simulink model "acoustic_pursuit_loop"  (R2026b)
settings: Solver=ode4  StopTime=30  FixedStep=0.01
model workspace (MAT data in the model file):
  Pc = [-0.955361961697; -8.18538892611e-15; -1.20667677978e-16; -0.534217529105; -8.61310855498e-16; -1.23431548867; -0.21823206593; -8.91503756517e-15; 0.05; 0; 0; -0.00125; 0; 0.25; 0.5; 0.523598775598; 0.145; 1; 1.3962634016; 0.1; 1; 0.05; 2.4; 0.03; 0.1]
  Po = [1; 0; 0; 0; 0; 0; 1; 0; 0; 0; 0; 0.125; 1; 0; 0; 0.05; 0; 0; 1; 0; 0; 0.003125; 0.05; 0; 1; -0.05; 0; 0; 0; 0; 0; -0.053125; -0.05; 0; 0; 1; 0; 0; 1; 0; 0; 0; 0; 0; 0; 0.878680113902; -3.59557130076e-18; 3.54139223511e-16; 0.51922603514; 7.21443661026e-16; -2.65527818364e-18; 0.970658487238; 1.08350382663; -8.10062906002e-17; 1.38781881493; 1; 0; 0; 0; 0; 0; 1; 0; 0; 0; 0; 0.75; 1; 0; 0; 0.3; 0; 0; 1; 0; 0; 0.1125; 0.3; 0; 1; 0.00370925831023; -5.96618963202e-20; -5.96618963197e-20; 0.0207679892018; 9.21; 0.15; 0.261799387799]
  Ps = [1; 1; 0.436332312999; 0.436332312999; 0.01; 0.05; 0.1; 0; 0.5; 0; 0; 5.6; 0.5]
  Td = 0.3
  Td_obs = 0.25
  Tdw = 0.1
  Tm = 0.4
  Ts = 0.05
  tau_v = 0.2
  tau_w = 0.15
  v0 = 0.25
  wt = [0.3; 0]
  x0 = [1.1; 0; 0]
settings Model: Creator=Admin  LastModifiedBy=Admin

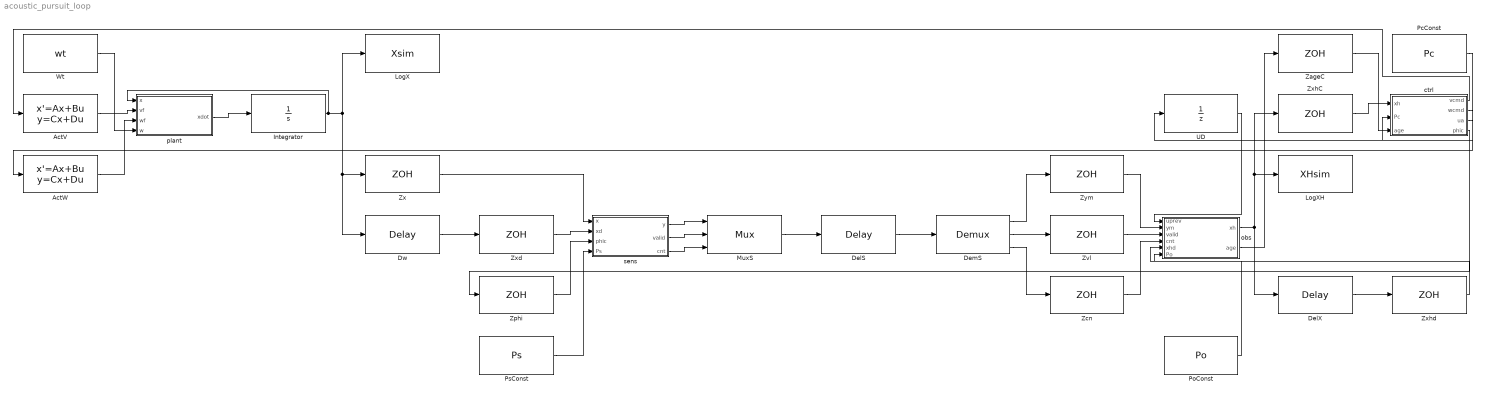
== system acoustic_pursuit_loop ==
  ActV : StateSpace  A=-1/tau_v  B=1/tau_v  D=0  InitialCondition=v0
  ActW : StateSpace  A=-1/tau_w  B=1/tau_w  D=0  InitialCondition=0
  DelS : TransportDelay  DelayTime=Td  InitialOutput=zeros(4,1)
  DelX : TransportDelay  DelayTime=Td_obs  InitialOutput=zeros(5,1)
  DemS : Demux  Outputs=[2 1 1]
  Dw : TransportDelay  DelayTime=Tdw  InitialOutput=x0
  Integrator : Integrator  InitialCondition=x0
  LogX : ToWorkspace  VariableName=Xsim  SampleTime=-1
  LogXH : ToWorkspace  VariableName=XHsim  SampleTime=-1
  MuxS : Mux  Inputs=3
  PcConst : Constant  Value=Pc
  PoConst : Constant  Value=Po
  PsConst : Constant  Value=Ps
  UD : UnitDelay  InitialCondition=[0;0]  SampleTime=Ts
  Wt : Constant  Value=wt
  ZageC : ZeroOrderHold  SampleTime=Ts
  Zcn : ZeroOrderHold  SampleTime=Ts
  Zphi : ZeroOrderHold  SampleTime=Tm
  Zvl : ZeroOrderHold  SampleTime=Ts
  Zx : ZeroOrderHold  SampleTime=Tm
  Zxd : ZeroOrderHold  SampleTime=Tm
  ZxhC : ZeroOrderHold  SampleTime=Ts
  Zxhd : ZeroOrderHold  SampleTime=Ts
  Zym : ZeroOrderHold  SampleTime=Ts
  ctrl : MATLAB Function  TreatAsAtomicUnit=on
  obs : MATLAB Function  TreatAsAtomicUnit=on
  plant : MATLAB Function  TreatAsAtomicUnit=on
  sens : MATLAB Function  TreatAsAtomicUnit=on
  wires:
  Wt/1 -> plant/4(w)
  ActV/1 -> plant/2(vf)
  ActW/1 -> plant/3(wf)
  Integrator/1 -> Zx/1, Dw/1, LogX/1, plant/1(x)
  plant/1(xdot) -> Integrator/1
  Zx/1 -> sens/1(x)
  Dw/1 -> Zxd/1
  Zxd/1 -> sens/2(xd)
  Zphi/1 -> sens/3(phic)
  PsConst/1 -> sens/4(Ps)
  sens/1(y) -> MuxS/1
  sens/2(valid) -> MuxS/2
  sens/3(cnt) -> MuxS/3
  MuxS/1 -> DelS/1
  DelS/1 -> DemS/1
  DemS/1 -> Zym/1
  DemS/2 -> Zvl/1
  DemS/3 -> Zcn/1
  Zym/1 -> obs/2(ym)
  Zvl/1 -> obs/3(valid)
  Zcn/1 -> obs/4(cnt)
  UD/1 -> obs/1(uprev)
  PoConst/1 -> obs/6(Po)
  obs/1(xh) -> LogXH/1, ZxhC/1, DelX/1
  DelX/1 -> Zxhd/1
  Zxhd/1 -> obs/5(xhd)
  ZxhC/1 -> ctrl/1(xh)
  PcConst/1 -> ctrl/2(Pc)
  obs/2(age) -> ZageC/1
  ZageC/1 -> ctrl/3(age)
  ctrl/1(vcmd) -> ActV/1
  ctrl/2(wcmd) -> ActW/1
  ctrl/3(ua) -> UD/1
  ctrl/4(phic) -> Zphi/1

== matlab function acoustic_pursuit_loop/sens ==
  data: x input; y output; xd input; phic input; Ps input; valid output; cnt output
function [y, valid, cnt] = sens(x, xd, phic, Ps)
% Paired acoustic measurement (Phase E): x at the A+ capture, xd at the A- capture (Tdw earlier).
% Multipath (Phase B s1): fast fringe = white ln-amplitude noise per capture (fr); room bias = AR(1) bearing bias
% (sd rsd, correlation time rtau) applied as A+/- * exp(+-b/(2h)). Same model as acoustic_pursuit_design.m sensor_pair.
persistent n room
if isempty(n), n = 0; room = 0; end
x = x(:); xd = xd(:); Ps = Ps(:);
K = Ps(1); Kerr = Ps(2); sig = Ps(3); dlt = Ps(4); sn = Ps(5); Athr = Ps(6); d = Ps(7); rp = Ps(8); rg = Ps(9);
fr = Ps(10); rsd = Ps(11); rtau = Ps(12); Tm = Ps(13);
if rsd > 0
    c = exp(-Tm/rtau);
    if n == 0, room = rsd*randn; else, room = c*room + sqrt(1 - c^2)*rsd*randn; end
end
h = sig^2/(2*dlt);
Am = amp_(K*Kerr, xd(1), xd(2), phic - dlt, sig, sn, rp, rg, fr)*exp(-room/(2*h));
Ap = amp_(K*Kerr, x(1),  x(2),  phic + dlt, sig, sn, rp, rg, fr)*exp(room/(2*h));
b = phic + sig^2/(2*dlt)*log(Ap/Am);
r = K/sqrt(Ap*Am)*exp(-((phic - b)^2 + dlt^2)/(2*sig^2));
y = [r - d; b];
valid = double(min(Am, Ap) > Athr);
n = n + 1;
cnt = n;

function A = amp_(Kt, rho, beta, phi, sig, sn, rp, rg, fr)
a0 = Kt/max(rho, 1e-2)*exp(-(phi - beta)^2/(2*sig^2));
if fr > 0, a0 = a0*exp(fr*randn); end
ec = complex(0,0);
if rp > 0 && rand < rp, ec = rg*a0*exp(1j*2*pi*rand); end
A = abs(complex(a0 + sn*randn, sn*randn) + ec);

== matlab function acoustic_pursuit_loop/plant ==
  data: x input; xdot output; vf input; wf input; w input
function xdot = plant(x, vf, wf, w)
x = x(:); w = w(:);
rho = max(x(1), 1e-2); beta = x(2); al = x(3) - beta;
xdot = [ w(1)*cos(al) - vf*cos(beta); ...
        (w(1)*sin(al) + vf*sin(beta))/rho - wf; ...
         w(2) - wf ];

== matlab function acoustic_pursuit_loop/obs ==
  data: uprev input; xh output; ym input; valid input; cnt input; xhd input; Po input; age output
function [xh, age] = obs(uprev, ym, valid, cnt, xhd, Po)
persistent x cprev init age_
if isempty(x), x = zeros(5,1); cprev = 0; init = false; age_ = 0; end
uprev = uprev(:); ym = ym(:); xhd = xhd(:); Po = Po(:);
Phi = reshape(Po(1:25),5,5); Gam = reshape(Po(26:35),5,2); Co = reshape(Po(36:45),2,5);
L = reshape(Po(46:55),5,2); PhiTd = reshape(Po(56:80),5,5);
S = reshape(Po(81:84),2,2); chi2 = Po(85); zr = Po(86); zb = Po(87);
x = Phi*x + Gam*uprev;
age_ = age_ + 1;
cn = round(cnt);
if abs(cnt - cn) < 1e-6 && cn ~= cprev          % clean sample only (Transport Delay may interpolate at edges)
    cprev = cn;
    if valid > 0.5
        if ~init
            x = PhiTd*[ym; 0; 0; 0];
            init = true;  age_ = 0;
        else
            nu = ym - Co*xhd;
            d2 = nu'*(S\nu);
            if abs(x(1)) < zr && abs(x(2)) < zb && d2 > chi2      % soft gate: clip the innovation, near lock only
                nu = nu*sqrt(chi2/d2);
            end
            x = x + PhiTd*(L*nu);  age_ = 0;
        end
    end
end
xh = x;
age = age_;

== matlab function acoustic_pursuit_loop/ctrl ==
  data: xh input; vcmd output; Pc input; age input; wcmd output; ua output; phic output
function [vcmd, wcmd, ua, phic] = ctrl(xh, Pc, age)
persistent z
if isempty(z), z = 0; end
xh = xh(:); Pc = Pc(:);
Kx = reshape(Pc(1:6),2,3); Kz = Pc(7:8); Ad4 = Pc(9:11).'; Bd4 = Pc(12:13).';
v0 = Pc(14); vmax = Pc(15); dsmax = Pc(16); Lw = Pc(17); zmax = Pc(18); phimax = Pc(19); zband = Pc(20); integ = Pc(21);
Ts = Pc(22); tlost = Pc(23); rstop = Pc(24); dstar = Pc(25);
stopped = (age*Ts > tlost) || (xh(1) + dstar < rstop);      % hard stop (watchdog)
u = -Kx*xh(1:3) - Kz*z;
vcmd = min(max(v0 + u(1), 0), vmax);
if stopped, vcmd = 0; end
wlim = max(vcmd, 0.05)*tan(dsmax)/Lw;
wcmd = min(max(u(2), -wlim), wlim);
if stopped, wcmd = 0; end
ua = [vcmd - v0; wcmd];
if integ > 0.5 && ~stopped && vcmd == v0 + u(1) && abs(xh(1)) < zband
    z = min(max(Ad4*xh(1:3) + z + Bd4*ua, -zmax), zmax);
end
phic = min(max(xh(2), -phimax), phimax);
